simulink model "PFC_Full_Bridge_IGBT_PR"  (R2021a)
settings: Solver=FixedStepAuto  StartTime=0.0  StopTime=2  RelTol=1e-3
InitFcn:
  | fsw = 50000;
  | Ts = 1/50000;
  | 
  | L = 680e-6;
  | C = 3660e-6;
  | 
  | Kpv = 0.393;
  | Kiv = 196.35;
  | 
  | Kpi = 21.4;
  | Kri = 85.6;
  | 
  | Ksogi = 1;
undefined symbols (not defined in the file or in its folder): DiscIntNeverNeededParam
libraries: spsIGBTDiodeLib x4, spsSeriesRLCBranchLib x4, spsCurrentMeasurementLib x2, spsMeanLib x2, pid_lib x2, simulink x2, spsRMSLib x2, spsVoltageMeasurementLib x2, spsACVoltageSourceLib x1, powerlib_extras x1, spsAlphaBetaZerotodq0Lib x1, spsTHDLib x1
settings Model: Creator=45276  LastModifiedBy=45276

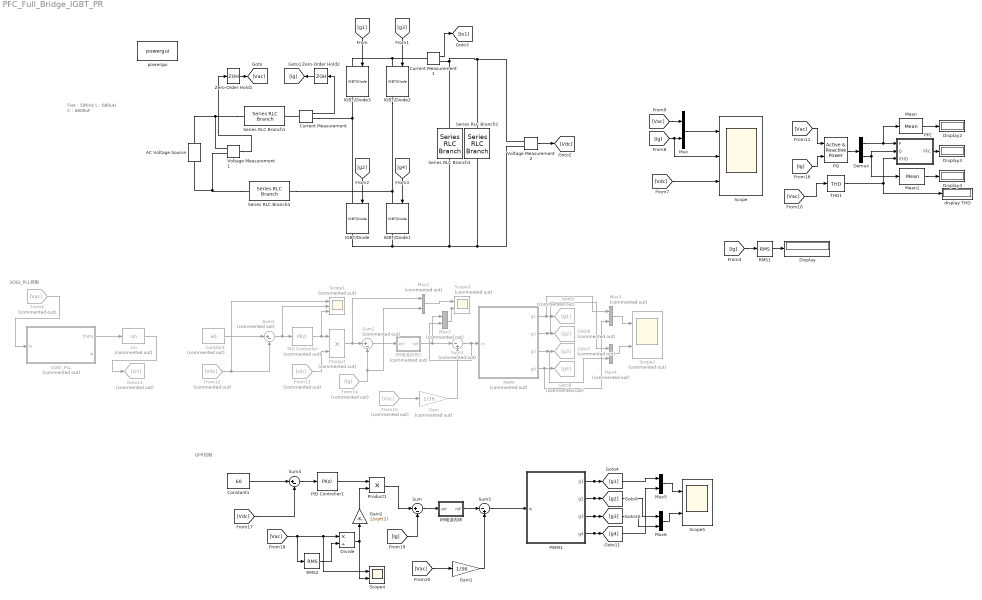
== system PFC_Full_Bridge_IGBT_PR ==
  note: Fsw：50KHz
      | L：680uH
      | C：6800uF
  note: SOGI_PLL控制
  note: QPR控制
  AC Voltage Source : spsACVoltageSourceLib/AC Voltage Source  Amplitude=36*sqrt(2)  Phase=0  Frequency=50  SampleTime=0  Measurements=None  BusType=swing  Pref=10e3  Qref=0  Qmin=-inf  Qmax=+inf
  Constant : Constant  Commented=on  Value=60
  Constant1 : Constant  Value=60
  Current Measurement : spsCurrentMeasurementLib/Current Measurement  PhasorSimulation=off  OutputType=Complex  PSBequivalent=0
  Current Measurement1 : spsCurrentMeasurementLib/Current Measurement  PhasorSimulation=off  OutputType=Complex  PSBequivalent=0
  Demux : Demux  Outputs=2
  Display{,2..4} (4 alike) : Display
  Divide : Product  Inputs=*/
  From12 : From  Commented=on  GotoTag=Vdc
  From13 : From  Commented=on  GotoTag=sin
  From14 : From  Commented=on  GotoTag=Ig
  From15 : From  Commented=on  GotoTag=Vac
  From6 : From  Commented=on  GotoTag=Vac
  Gain : Gain  Commented=on  Gain=1/36
  Gain1 : Gain  Gain=1/36
  Gain2 : Gain  Gain=1/sqrt(2)
  Goto13 : Goto  Commented=on  GotoTag=sin
  Goto5 : Goto  Commented=on  GotoTag=g1
  Goto6 : Goto  Commented=on  GotoTag=g2
  Goto7 : Goto  Commented=on  GotoTag=g3
  Goto8 : Goto  Commented=on  GotoTag=g4
  IGBT/Diode{,1..3} (4 alike) : spsIGBTDiodeLib/IGBT//Diode  Ron=1e-3  Rs=1e5  Cs=inf  Measurements=on
  Mean : spsMeanLib/Mean  Freq=50  Vinit=0  Ts=0
  Mean1 : spsMeanLib/Mean  Freq=50  Vinit=0  Ts=0
  Mux : Mux  Inputs=2
  Mux{1..4} (4 alike) : Mux  Commented=on  Inputs=2
  Mux5 : Mux  Inputs=2
  Mux6 : Mux  Inputs=2
  PFC : MATLAB Function  TreatAsAtomicUnit=on
  PID Controller : pid_lib/PID Controller  Commented=on  Controller=PI  Form=Parallel  TimeDomain=Discrete-time  UseExternalTs=off  SampleTime=Ts  IntegratorMethod=Trapezoidal  FilterMethod=Forward Euler  ControllerParametersSource=internal  P=Kpv  I=Kiv  D=0  UseFilter=on  N=100  TunerSelectOption=Transfer Function Based (PID Tuner App)  InitialConditionSource=internal  InitialConditionForIntegrator=0  InitialConditionForFilter=0  DifferentiatorICPrevScaledInput=0  ExternalReset=none  TrackingMode=off  Kt=1  LimitOutput=off  SatLimitsSource=internal  UpperSaturationLimit=inf  LowerSaturationLimit=-inf  LinearizeAsGain=on  AntiWindupMode=none  Kb=1  POutMin=[]  POutMax=[]  IOutMin=[]  IOutMax=[]  DOutMin=[]  DOutMax=[]  NOutMin=[]  NOutMax=[]  SumOutMin=[]  SumOutMax=[]  SaturationOutMin=[]  SaturationOutMax=[]  PParamMin=[]  PParamMax=[]  IParamMin=[]  IParamMax=[]  DParamMin=[]  DParamMax=[]  NParamMin=[]  NParamMax=[]  KbParamMin=[]  KbParamMax=[]  KtParamMin=[]  KtParamMax=[]  KbOutMin=[]  KbOutMax=[]  KtOutMin=[]  KtOutMax=[]  IntegratorOutMin=[]  IntegratorOutMax=[]  FilterOutMin=[]  FilterOutMax=[]  SumI1OutMin=[]  SumI1OutMax=[]  SumI2OutMin=[]  SumI2OutMax=[]  SumI3OutMin=[]  SumI3OutMax=[]  SumI4OutMin=[]  SumI4OutMax=[]  SumDOutMin=[]  SumDOutMax=[]  DifferentiatorOutMin=[]  DifferentiatorOutMax=[]  FilterDiffOutCoefMin=[]  FilterDiffOutCoefMax=[]  ReciprocalOutMin=[]  ReciprocalOutMax=[]  SumDenOutMin=[]  SumDenOutMax=[]  SumNumOutMin=[]  SumNumOutMax=[]  DivideOutMin=[]  DivideOutMax=[]  UdiffTsProdOutMin=[]  UdiffTsProdOutMax=[]  NTsProdOutMin=[]  NTsProdOutMax=[]  UintegralTsProdOutMin=[]  UintegralTsProdOutMax=[]  UngainTsProdOutMin=[]  UngainTsProdOutMax=[]  IntegratorContinuousStateAttributes=''  IntegratorStateMustResolveToSignalObject=off  IntegratorRTWStateStorageClass=Auto  FilterContinuousStateAttributes=''  FilterStateMustResolveToSignalObject=off  FilterRTWStateStorageClass=Auto  ParallelPVariant=InternalParameters  IdealPVariant=Disabled  IVariant=InternalParameters  DVariant=Disabled  IntegratorVariant=Discrete  SatVariant=Disabled  AWVariant=Passthrough  PCopyVariant=Disabled  TRVariant=Disabled  FdbkBlocksVariant=Forward  IdealPFdbkVariant=Disabled  SatFdbkVariant=Disabled  DerivativeFilterVariant=Disabled  NVariant=Disabled  NCopyVariant=Disabled_SignalSpec  FilterICVariant=Disabled  IntegratorICVariant=InternalICs  ExternalResetVariant=Disabled  TRSumVariant=Passthrough  SumFdbkVariant=Disabled  SumVariant=Sum_PI  TsampFilterVariant=InternalTs  TsampNgainVariant=Passthrough  TsampIntegralVariant=Passthrough  ExternalSaturationOutDataTypeStr=Inherit: Same as second input
  PID Controller1 : pid_lib/PID Controller  Controller=PI  Form=Parallel  TimeDomain=Discrete-time  UseExternalTs=off  SampleTime=Ts  IntegratorMethod=Trapezoidal  FilterMethod=Forward Euler  ControllerParametersSource=internal  P=Kpv  I=Kiv  D=0  UseFilter=on  N=100  TunerSelectOption=Transfer Function Based (PID Tuner App)  InitialConditionSource=internal  InitialConditionForIntegrator=0  InitialConditionForFilter=0  DifferentiatorICPrevScaledInput=0  ExternalReset=none  TrackingMode=off  Kt=1  LimitOutput=off  SatLimitsSource=internal  UpperSaturationLimit=inf  LowerSaturationLimit=-inf  LinearizeAsGain=on  AntiWindupMode=none  Kb=1  POutMin=[]  POutMax=[]  IOutMin=[]  IOutMax=[]  DOutMin=[]  DOutMax=[]  NOutMin=[]  NOutMax=[]  SumOutMin=[]  SumOutMax=[]  SaturationOutMin=[]  SaturationOutMax=[]  PParamMin=[]  PParamMax=[]  IParamMin=[]  IParamMax=[]  DParamMin=[]  DParamMax=[]  NParamMin=[]  NParamMax=[]  KbParamMin=[]  KbParamMax=[]  KtParamMin=[]  KtParamMax=[]  KbOutMin=[]  KbOutMax=[]  KtOutMin=[]  KtOutMax=[]  IntegratorOutMin=[]  IntegratorOutMax=[]  FilterOutMin=[]  FilterOutMax=[]  SumI1OutMin=[]  SumI1OutMax=[]  SumI2OutMin=[]  SumI2OutMax=[]  SumI3OutMin=[]  SumI3OutMax=[]  SumI4OutMin=[]  SumI4OutMax=[]  SumDOutMin=[]  SumDOutMax=[]  DifferentiatorOutMin=[]  DifferentiatorOutMax=[]  FilterDiffOutCoefMin=[]  FilterDiffOutCoefMax=[]  ReciprocalOutMin=[]  ReciprocalOutMax=[]  SumDenOutMin=[]  SumDenOutMax=[]  SumNumOutMin=[]  SumNumOutMax=[]  DivideOutMin=[]  DivideOutMax=[]  UdiffTsProdOutMin=[]  UdiffTsProdOutMax=[]  NTsProdOutMin=[]  NTsProdOutMax=[]  UintegralTsProdOutMin=[]  UintegralTsProdOutMax=[]  UngainTsProdOutMin=[]  UngainTsProdOutMax=[]  IntegratorContinuousStateAttributes=''  IntegratorStateMustResolveToSignalObject=off  IntegratorRTWStateStorageClass=Auto  FilterContinuousStateAttributes=''  FilterStateMustResolveToSignalObject=off  FilterRTWStateStorageClass=Auto  ParallelPVariant=InternalParameters  IdealPVariant=Disabled  IVariant=InternalParameters  DVariant=Disabled  IntegratorVariant=Discrete  SatVariant=Disabled  AWVariant=Passthrough  PCopyVariant=Disabled  TRVariant=Disabled  FdbkBlocksVariant=Forward  IdealPFdbkVariant=Disabled  SatFdbkVariant=Disabled  DerivativeFilterVariant=Disabled  NVariant=Disabled  NCopyVariant=Disabled_SignalSpec  FilterICVariant=Disabled  IntegratorICVariant=InternalICs  ExternalResetVariant=Disabled  TRSumVariant=Passthrough  SumFdbkVariant=Disabled  SumVariant=Sum_PI  TsampFilterVariant=InternalTs  TsampNgainVariant=Passthrough  TsampIntegralVariant=Passthrough  ExternalSaturationOutDataTypeStr=Inherit: Same as second input
  PQ : powerlib_extras/Measurements/Active & Reactive Power  f1=50
      settings: SourceProductBaseCode=PS
  PR电流内环 : Subsystem  TreatAsAtomicUnit=on  mask{Kp=Kpi, Kr=Kri, Wc=5, Upper=200, Lower=-200}
  PR电流内环1 : Subsystem  Commented=on  TreatAsAtomicUnit=on  mask{Kp=Kpi, Kr=Kri, Wc=5, Upper=200, Lower=-200}
  PWM : Subsystem  Commented=on
  PWM1 : Subsystem
  Product : Product  Commented=on
  Product1 : Product
  RMS1 : spsRMSLib/RMS  TrueRMS=on  Freq=60  RMSInit=120  Ts=0
  RMS2 : spsRMSLib/RMS  TrueRMS=on  Freq=60  RMSInit=120  Ts=0
  SOGI_PLL : Subsystem  Commented=on
  Scope : Scope  NumInputPorts=3
  Scope1 : Scope  Commented=on  NumInputPorts=3
  Scope2 : Scope  Commented=on  NumInputPorts=2
  Scope3 : Scope  Commented=on  NumInputPorts=2
  Scope4 : Scope  NumInputPorts=2
  Scope5 : Scope  NumInputPorts=2
  Series RLC Branch1 : spsSeriesRLCBranchLib/Series RLC Branch  LConnTagsString=__new0  RConnTagsString=__new0  BranchType=RL  Resistance=0.1  Inductance=L  SetiL0=off  InitialCurrent=0  Capacitance=1e-6  Setx0=off  InitialVoltage=0  Measurements=None
  Series RLC Branch2 : spsSeriesRLCBranchLib/Series RLC Branch  LConnTagsString=__new0  RConnTagsString=__new0  BranchType=RL  Resistance=20  Inductance=1e-9  SetiL0=off  InitialCurrent=0  Capacitance=C  Setx0=off  InitialVoltage=0  Measurements=None
  Series RLC Branch3 : spsSeriesRLCBranchLib/Series RLC Branch  LConnTagsString=__new0  RConnTagsString=__new0  BranchType=RC  Resistance=0.25  Inductance=1e-3  SetiL0=off  InitialCurrent=0  Capacitance=C  Setx0=off  InitialVoltage=0  Measurements=None
  Series RLC Branch4 : spsSeriesRLCBranchLib/Series RLC Branch  LConnTagsString=__new0  RConnTagsString=__new0  BranchType=RL  Resistance=0.1  Inductance=L  SetiL0=off  InitialCurrent=0  Capacitance=1e-6  Setx0=off  InitialVoltage=0  Measurements=None
  Sum : Sum  Inputs=|+-
  Sum1 : Sum  Commented=on  Inputs=|+-
  Sum2 : Sum  Commented=on  Inputs=|+-
  Sum3 : Sum  Commented=on  Inputs=|-+
  Sum4 : Sum  Inputs=|+-
  Sum5 : Sum  Inputs=|-+
  THD1 : spsTHDLib/THD  Freq=60  Ts=0
      settings: SourceProductBaseCode=PS
  Voltage Measurement1 : spsVoltageMeasurementLib/Voltage Measurement  PhasorSimulation=off  OutputType=Complex  PSBequivalent=0
  Voltage Measurement2 : spsVoltageMeasurementLib/Voltage Measurement  PhasorSimulation=off  OutputType=Complex  PSBequivalent=0
  Zero-Order Hold1 : ZeroOrderHold  SampleTime=Ts
  Zero-Order Hold2 : ZeroOrderHold  SampleTime=Ts
  display THD : Display
  powergui : spspowerguiLib/powergui  Priority=1  SimulationMode=Discrete  SampleTime=1e-6  frequency=60  Iterations=50  frequencyindice=50  Pbase=100e6  ErrMax=1e-4  UnitsV=kV  UnitsW=MW  buscounter=0  FunctionMessages=off  echomessages=off  EnableUseOfTLC=off  CurrentSourceSwitches=off  DisableSnubberDevices=off  DisableRonSwitches=off  DisableVfSwitches=off  DisplayEquations=off  AutomaticDiscreteSolvers=off  SolverType=Tustin/Backward Euler (TBE)  Interpol=off  ExternalGateDelay=off  methode=off  Ts=100  x0status=blocks  SPID=on  SwTol=0  HookPort=off  NonlinearTolerance=1e-4  nMaxIteration=100  ContinueOnMaxIteration=off  RestoreLinks=warning  ResistiveCurrentMeasurement=off  Frange=[0:2:500]  Ylog=off  Xlog=on  ShowGrid=off  save=off  variable=ZData  structure=0  ZoomFFT=off  StartTime=0.0  cycles=1  DisplayStyle=1  fundamental=60  FreqAxis=off  MaxFrequency=1000  frequencyindicesteady=1  RmsSteady=1  display=off
  sin : Trigonometry  Commented=on
  wires:
  Voltage Measurement1/1 -> Zero-Order Hold1/1
  Zero-Order Hold2/1 -> [Ig]
  [g1] -> IGBT/Diode3/1
  [g2] -> IGBT/Diode/1
  [g3] -> IGBT/Diode2/1
  [g4] -> IGBT/Diode1/1
  Current Measurement1/1 -> [Io1]
  Zero-Order Hold1/1 -> [Vac]
  Current Measurement/1 -> Zero-Order Hold2/1
  PWM/1(g1) -> Mux3/1, Goto5/1
  From13/1 -> Product/2
  PWM/2(g2) -> Mux4/1, Goto6/1
  PWM/3(g3) -> Mux4/2, Goto7/1
  Mux1/1 -> Scope3/1
  From12/1 -> Sum1/2, Scope1/1
  PID Controller/1 -> Product/1, Scope1/3
  Gain/1 -> Sum3/2
  Sum1/1 -> Scope1/2, PID Controller/1
  From14/1 -> Mux1/2, Sum2/2
  Sum3/1 -> Mux2/2, PWM/1(in)
  Sum2/1 -> PR电流内环1/1(err)
  Mux2/1 -> Scope3/2
  From15/1 -> Gain/1
  Product/1 -> Mux1/1, Sum2/1
  Constant/1 -> Sum1/1
  PWM/4(g4) -> Mux3/2, Goto8/1
  PR电流内环1/1(ref) -> Mux2/1, Sum3/1
  SOGI_PLL/1(theta) -> sin/1
  From6/1 -> SOGI_PLL/1(in)
  sin/1 -> Goto13/1
  Voltage Measurement2/1 -> [Vdc]
  [Ig] -> RMS1/1
  Mux/1 -> Scope/1
  [Ig] -> Scope/2, Mux/2
  [Vac] -> Mux/1
  [Vdc] -> Scope/3
  Mux3/1 -> Scope2/1
  Mux4/1 -> Scope2/2
  PQ/1 -> Demux/1
  Demux/1 -> Mean/1, PFC/1(P)
  Demux/2 -> PFC/2(Q), Mean1/1
  Mean1/1 -> Display4/1
  PFC/1(PFC) -> Display3/1
  THD1/1 -> PFC/3(iTHD), display THD/1
  [Vac] -> THD1/1
  [Vac] -> PQ/1
  [Ig] -> PQ/2
  Mean/1 -> Display2/1
  RMS2/1 -> Divide/2
  Divide/1 -> Gain2/1, Scope4/2
  Mux5/1 -> Scope5/1
  PWM1/2(g2) -> Mux6/1, [g2]
  [Vdc] -> Sum4/2
  Constant1/1 -> Sum4/1
  PWM1/1(g1) -> Mux5/1, [g1]
  Sum/1 -> PR电流内环/1(err)
  Sum4/1 -> PID Controller1/1
  Mux6/1 -> Scope5/2
  PWM1/3(g3) -> Mux6/2, [g3]
  PWM1/4(g4) -> Mux5/2, [g4]
  [Vac] -> RMS2/1, Scope4/1, Divide/1
  [Ig] -> Sum/2
  PID Controller1/1 -> Product1/1
  RMS1/1 -> Display/1
  [Vac] -> Gain1/1
  Gain1/1 -> Sum5/2
  PR电流内环/1(ref) -> Sum5/1
  Sum5/1 -> PWM1/1(in)
  Product1/1 -> Sum/1
  Gain2/1 -> Product1/2
  connections:
  Current Measurement1/RConn1 -- Series RLC Branch2/LConn1 -- Voltage Measurement2/LConn1 -- Series RLC Branch3/LConn1
  IGBT/Diode3/LConn1 -- IGBT/Diode2/LConn1 -- Current Measurement1/LConn1
  Series RLC Branch4/LConn1 -- Voltage Measurement1/LConn2 -- AC Voltage Source/LConn1
  Series RLC Branch1/LConn1 -- AC Voltage Source/RConn1 -- Voltage Measurement1/LConn1
  IGBT/Diode3/RConn1 -- IGBT/Diode/LConn1 -- Current Measurement/RConn1
  Current Measurement/LConn1 -- Series RLC Branch1/RConn1
  IGBT/Diode1/RConn1 -- IGBT/Diode/RConn1 -- Series RLC Branch2/RConn1 -- Voltage Measurement2/LConn2 -- Series RLC Branch3/RConn1
  Series RLC Branch4/RConn1 -- IGBT/Diode2/RConn1 -- IGBT/Diode1/LConn1

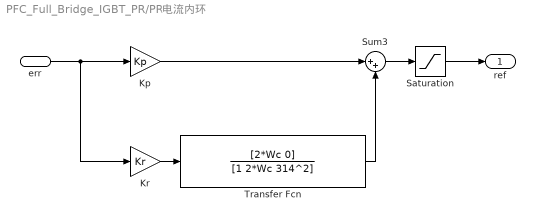
== system PFC_Full_Bridge_IGBT_PR/PR电流内环 ==
  err : Inport
  Kp : Gain  Gain=Kp
  Kr : Gain  Gain=Kr
  Saturation : Saturate  UpperLimit=Upper  LowerLimit=Lower
  Sum3 : Sum  Inputs=|++
  Transfer Fcn : TransferFcn  Numerator=[2*Wc 0]  Denominator=[1 2*Wc 314^2]
  ref : Outport
  wires:
  Kp/1 -> Sum3/1
  Sum3/1 -> Saturation/1
  err/1 -> Kr/1, Kp/1
  Kr/1 -> Transfer Fcn/1
  Transfer Fcn/1 -> Sum3/2
  Saturation/1 -> ref/1

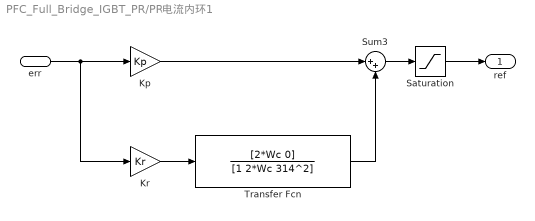
== system PFC_Full_Bridge_IGBT_PR/PR电流内环1 ==
  err : Inport
  Kp : Gain  Gain=Kp
  Kr : Gain  Gain=Kr
  Saturation : Saturate  UpperLimit=Upper  LowerLimit=Lower
  Sum3 : Sum  Inputs=|++
  Transfer Fcn : TransferFcn  Numerator=[2*Wc 0]  Denominator=[1 2*Wc 314^2]
  ref : Outport
  wires:
  Saturation/1 -> ref/1
  Transfer Fcn/1 -> Sum3/2
  Kr/1 -> Transfer Fcn/1
  err/1 -> Kp/1, Kr/1
  Sum3/1 -> Saturation/1
  Kp/1 -> Sum3/1

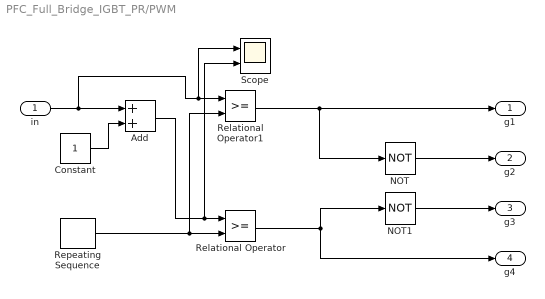
== system PFC_Full_Bridge_IGBT_PR/PWM ==
  in : Inport
  Add : Sum
  Constant : Constant
  NOT : Logic  Operator=NOT  IconShape=distinctive  AllPortsSameDT=off  OutDataTypeStr=boolean
  NOT1 : Logic  Operator=NOT  IconShape=distinctive  AllPortsSameDT=off  OutDataTypeStr=boolean
  Relational Operator : RelationalOperator  OutDataTypeStr=boolean  RndMeth=Simplest
  Relational Operator1 : RelationalOperator  OutDataTypeStr=boolean  RndMeth=Simplest
  Repeating Sequence : simulink/Sources/Repeating Sequence  rep_seq_t=[0 Ts/2 Ts]  rep_seq_y=[0 1 0]
  Scope : Scope  NumInputPorts=2
  g1 : Outport
  g2 : Outport  Port=2
  g3 : Outport  Port=3
  g4 : Outport  Port=4
  wires:
  Add/1 -> Scope/2, Relational Operator/1
  Constant/1 -> Add/2
  Relational Operator1/1 -> g1/1, NOT/1
  Relational Operator/1 -> g4/1, NOT1/1
  NOT/1 -> g2/1
  in/1 -> Scope/1, Relational Operator1/1, Add/1
  NOT1/1 -> g3/1
  Repeating Sequence/1 -> Relational Operator1/2, Relational Operator/2

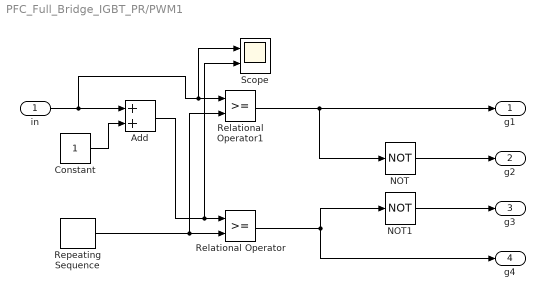
== system PFC_Full_Bridge_IGBT_PR/PWM1 ==
  in : Inport
  Add : Sum
  Constant : Constant
  NOT : Logic  Operator=NOT  IconShape=distinctive  AllPortsSameDT=off  OutDataTypeStr=boolean
  NOT1 : Logic  Operator=NOT  IconShape=distinctive  AllPortsSameDT=off  OutDataTypeStr=boolean
  Relational Operator : RelationalOperator  OutDataTypeStr=boolean  RndMeth=Simplest
  Relational Operator1 : RelationalOperator  OutDataTypeStr=boolean  RndMeth=Simplest
  Repeating Sequence : simulink/Sources/Repeating Sequence  rep_seq_t=[0 Ts/2 Ts]  rep_seq_y=[0 1 0]
  Scope : Scope  NumInputPorts=2
  g1 : Outport
  g2 : Outport  Port=2
  g3 : Outport  Port=3
  g4 : Outport  Port=4
  wires:
  Add/1 -> Scope/2, Relational Operator/1
  Constant/1 -> Add/2
  Relational Operator1/1 -> g1/1, NOT/1
  Relational Operator/1 -> g4/1, NOT1/1
  NOT/1 -> g2/1
  in/1 -> Scope/1, Relational Operator1/1, Add/1
  NOT1/1 -> g3/1
  Repeating Sequence/1 -> Relational Operator1/2, Relational Operator/2

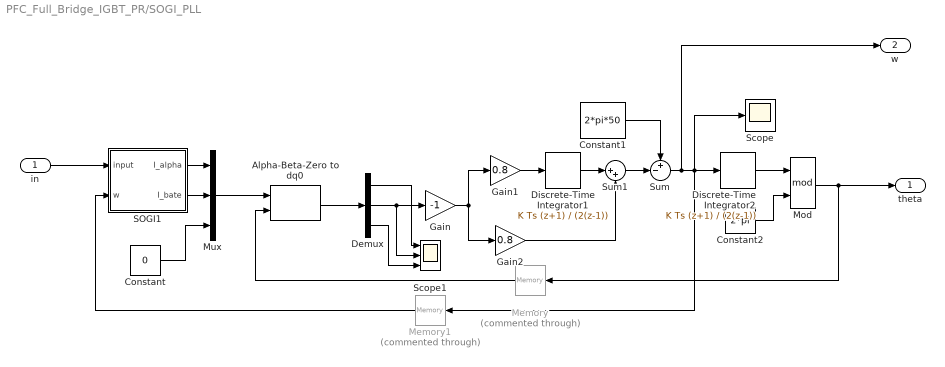
== system PFC_Full_Bridge_IGBT_PR/SOGI_PLL ==
  in : Inport
  Alpha-Beta-Zero to dq0 : spsAlphaBetaZerotodq0Lib/Alpha-Beta-Zero to dq0  Alignment=90 degrees behind phase A axis
      settings: SourceProductBaseCode=PS
  Constant : Constant  Value=0
  Constant1 : Constant  Value=2*pi*50
  Constant2 : Constant  Value=2*pi
  Demux : Demux  Outputs=3
  Discrete-Time Integrator1 : DiscreteIntegrator  IntegratorMethod=Integration: Trapezoidal  SampleTime=Ts  ICPrevOutput=DiscIntNeverNeededParam  ICPrevScaledInput=DiscIntNeverNeededParam
  Discrete-Time Integrator2 : DiscreteIntegrator  IntegratorMethod=Integration: Trapezoidal  SampleTime=Ts  ICPrevOutput=DiscIntNeverNeededParam  ICPrevScaledInput=DiscIntNeverNeededParam
  Gain : Gain  Gain=-1
  Gain1 : Gain  Gain=0.8
  Gain2 : Gain  Gain=0.8
  Memory : Memory  Commented=through
  Memory1 : Memory  Commented=through
  Mod : Math  Operator=mod  SaturateOnIntegerOverflow=on
  Mux : Mux  Inputs=3
  SOGI1 : Subsystem
  Scope : Scope
  Scope1 : Scope  NumInputPorts=3
  Sum : Sum  Inputs=+-|
  Sum1 : Sum  Inputs=|++
  theta : Outport
  w : Outport  Port=2
  wires:
  Demux/2 -> Gain/1, Scope1/2
  Sum/1 -> w/1, Memory1/1, Scope/1, Discrete-Time Integrator2/1
  Gain2/1 -> Sum1/2
  Alpha-Beta-Zero to dq0/1 -> Demux/1
  Mod/1 -> theta/1, Memory/1
  Discrete-Time Integrator1/1 -> Sum1/1
  Gain/1 -> Gain2/1, Gain1/1
  Mux/1 -> Alpha-Beta-Zero to dq0/1
  Discrete-Time Integrator2/1 -> Mod/1
  SOGI1/2(I_bate) -> Mux/2
  Memory/1 -> Alpha-Beta-Zero to dq0/2
  Constant2/1 -> Mod/2
  in/1 -> SOGI1/1(input)
  Memory1/1 -> SOGI1/2(w)
  Sum1/1 -> Sum/2
  SOGI1/1(I_alpha) -> Mux/1
  Constant1/1 -> Sum/1
  Gain1/1 -> Discrete-Time Integrator1/1
  Constant/1 -> Mux/3
  Demux/3 -> Scope1/3
  Demux/1 -> Scope1/1

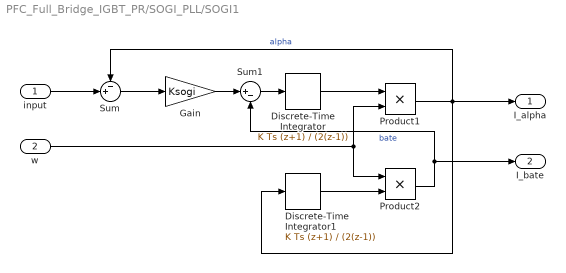
== system PFC_Full_Bridge_IGBT_PR/SOGI_PLL/SOGI1 ==
  input : Inport
  w : Inport  Port=2
  Discrete-Time Integrator : DiscreteIntegrator  IntegratorMethod=Integration: Trapezoidal  SampleTime=Ts  ICPrevOutput=DiscIntNeverNeededParam  ICPrevScaledInput=DiscIntNeverNeededParam
  Discrete-Time Integrator1 : DiscreteIntegrator  IntegratorMethod=Integration: Trapezoidal  SampleTime=Ts  ICPrevOutput=DiscIntNeverNeededParam  ICPrevScaledInput=DiscIntNeverNeededParam
  Gain : Gain  Gain=Ksogi
  Product1 : Product
  Product2 : Product
  Sum : Sum  Inputs=-+|
  Sum1 : Sum  Inputs=|+-
  I_alpha : Outport
  I_bate : Outport  Port=2
  wires:
  Sum1/1 -> Discrete-Time Integrator/1
  w/1 -> Product1/2, Product2/1
  Discrete-Time Integrator1/1 -> Product2/2
  Product2/1 -> I_bate/1, Sum1/2  "bate"
  Product1/1 -> I_alpha/1, Sum/1, Discrete-Time Integrator1/1  "alpha"
  input/1 -> Sum/2
  Sum/1 -> Gain/1
  Gain/1 -> Sum1/1
  Discrete-Time Integrator/1 -> Product1/1

== matlab function PFC_Full_Bridge_IGBT_PR/PFC ==
  data: P input; PFC output; Q input; iTHD input
function PFC = fcn(P,Q,iTHD)
% This block supports an embeddable subset of the MATLAB language.
% See the help menu for details. 
PFC=(P/sqrt(P*P+Q*Q))/sqrt(1+iTHD^2);
